simulink model "chopper_prototype_rating"  (R2024b)
settings: Solver=ode23tb  StartTime=0.0  StopTime=1  MaxStep=1e-4  RelTol=1e-3
libraries: spsDCVoltageSourceLib x2, spsDiodeLib x2, spsMosfetLib x2, spsCurrentMeasurementLib x1, spsMeanLib x1, spsSeriesRLCBranchLib x1, spsVoltageMeasurementLib x1, sps_lib x1
settings Model: Creator=Parti  LastModifiedBy=Eng.Abd-Elrhman Saad

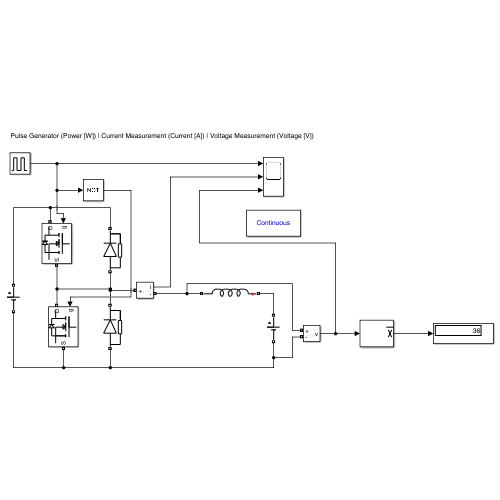
[thumbnail: Simulink's stored preview of the top-level diagram]
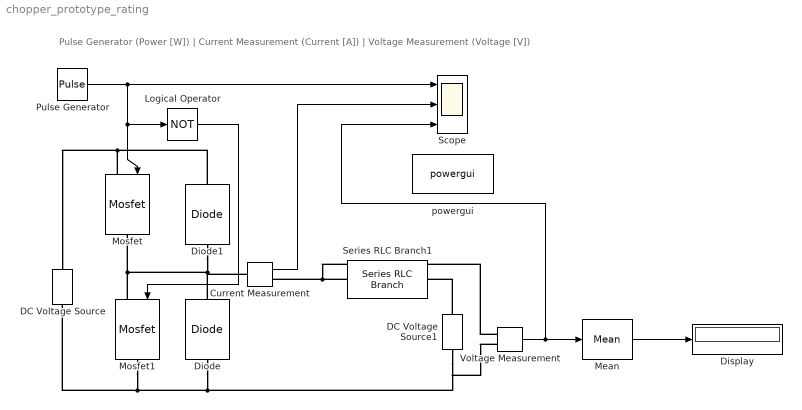
== system chopper_prototype_rating ==
  note: Pulse Generator (Power [W]) | Current Measurement (Current [A]) | Voltage Measurement (Voltage [V])
  Current Measurement : spsCurrentMeasurementLib/Current Measurement  PhasorSimulation=off  OutputType=Complex  PSBequivalent=0
  DC Voltage Source : spsDCVoltageSourceLib/DC Voltage Source  Amplitude=48  Measurements=None
  DC Voltage Source1 : spsDCVoltageSourceLib/DC Voltage Source  Amplitude=36  Measurements=None
  Diode : spsDiodeLib/Diode  Ron=0.001  Lon=0  Vf=0.8  IC=0  UseSnubber=0  Rs=500  Cs=250e-9  Measurements=off
  Diode1 : spsDiodeLib/Diode  Ron=0.001  Lon=0  Vf=0.8  IC=0  UseSnubber=0  Rs=500  Cs=250e-9  Measurements=off
  Display : Display
  Logical Operator : Logic  Operator=NOT  Inputs=3  AllPortsSameDT=off  OutDataTypeStr=boolean
  Mean : spsMeanLib/Mean  Freq=50  Vinit=0  Ts=0
  Mosfet : spsMosfetLib/Mosfet  Ron=0.1  Lon=0  Rd=0.01  Vfd=0  IC=0  Rs=1e5  Cs=inf  Measurements=off
  Mosfet1 : spsMosfetLib/Mosfet  Ron=0.1  Lon=0  Rd=0.01  Vfd=0  IC=0  Rs=1e5  Cs=inf  Measurements=off
  Pulse Generator : DiscretePulseGenerator  PulseType=Time based  Amplitude=10  Period=5e-5  PulseWidth=75
  Scope : Scope  NumInputPorts=3
  Series RLC Branch1 : spsSeriesRLCBranchLib/Series RLC Branch  LConnTagsString=__new0  RConnTagsString=__new0  BranchType=L  Resistance=10  Inductance=4.5e-4  SetiL0=off  InitialCurrent=0  Capacitance=1e-6  Setx0=off  InitialVoltage=0  Measurements=None
  Voltage Measurement : spsVoltageMeasurementLib/Voltage Measurement  PhasorSimulation=off  OutputType=Complex  PSBequivalent=0
  powergui : sps_lib/powergui  Priority=1  SimulationMode=Continuous  SampleTime=50e-6  frequency=60  Iterations=50  frequencyindice=0  Pbase=100e6  ErrMax=1e-4  UnitsV=kV  UnitsW=MW  buscounter=0  FunctionMessages=off  echomessages=off  EnableUseOfTLC=off  CurrentSourceSwitches=off  DisableSnubberDevices=off  DisableRonSwitches=off  DisableVfSwitches=off  DisplayEquations=off  AutomaticDiscreteSolvers=off  SolverType=Tustin/Backward Euler (TBE)  Interpol=off  ExternalGateDelay=off  methode=off  Ts=100  x0status=blocks  SPID=on  SwTol=0  HookPort=off  NonlinearTolerance=1e-4  nMaxIteration=100  ContinueOnMaxIteration=off  RestoreLinks=warning  ResistiveCurrentMeasurement=off  Frange=[0:2:500]  Ylog=off  Xlog=on  ShowGrid=off  save=off  variable=ZData  structure=0  ZoomFFT=off  StartTime=0.0  cycles=1  DisplayStyle=1  fundamental=60  FreqAxis=off  MaxFrequency=1000  frequencyindicesteady=1  RmsSteady=1  display=off
  wires:
  Pulse Generator/1 -> Scope/1, Mosfet/1, Logical Operator/1
  Logical Operator/1 -> Mosfet1/1
  Voltage Measurement/1 -> Scope/3, Mean/1
  Mean/1 -> Display/1
  Current Measurement/1 -> Scope/2
  connections:
  Mosfet1/RConn1 -- Voltage Measurement/LConn2 -- DC Voltage Source1/LConn1 -- Diode/LConn1 -- DC Voltage Source/LConn1
  DC Voltage Source1/RConn1 -- Series RLC Branch1/LConn1
  Mosfet1/LConn1 -- Diode/RConn1 -- Current Measurement/LConn1 -- Diode1/LConn1 -- Mosfet/RConn1
  Mosfet/LConn1 -- Diode1/RConn1 -- DC Voltage Source/RConn1
  Series RLC Branch1/RConn1 -- Voltage Measurement/LConn1 -- Current Measurement/RConn1
